simulink subsystem "DCM2quat"  (R2024b)
settings: Solver=VariableStepAuto  StartTime=0.0  StopTime=10.0  RelTol=1e-3
libraries: simulink x2
settings Model: Creator=ferru  LastModifiedBy=domac

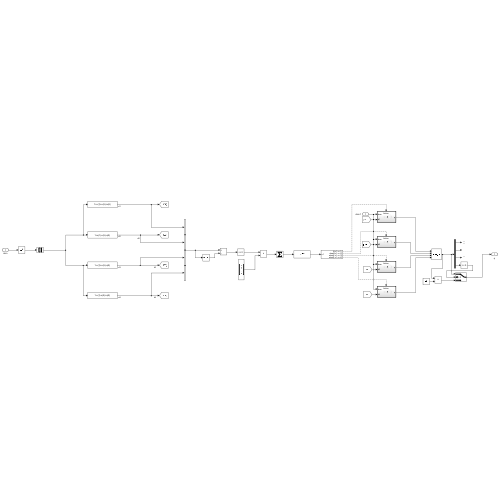
[thumbnail: Simulink's stored preview of the top-level diagram]
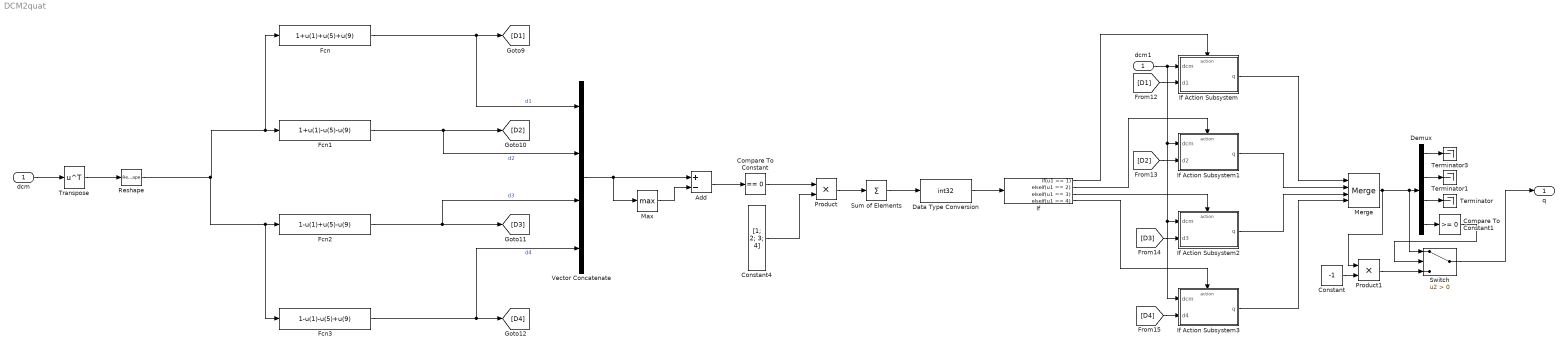
== system DCM2quat ==
  dcm : Inport
  Add : Sum  Inputs=+-
  Compare To Constant : simulink/Logic and Bit Operations/Compare To Constant  relop===  const=0  OutDataTypeStr=boolean
  Compare To Constant1 : simulink/Logic and Bit Operations/Compare To Constant  relop=>=  const=0  OutDataTypeStr=boolean
  Constant : Constant  Value=-1
  Constant4 : Constant  Value=[1; 2; 3; 4]  VectorParams1D=off
  Data Type Conversion : DataTypeConversion  OutDataTypeStr=int32  RndMeth=Round  SaturateOnIntegerOverflow=off
  Demux : Demux
  Fcn : Fcn  Expr=1+u(1)+u(5)+u(9)
  Fcn1 : Fcn  Expr=1+u(1)-u(5)-u(9)
  Fcn2 : Fcn  Expr=1-u(1)+u(5)-u(9)
  Fcn3 : Fcn  Expr=1-u(1)-u(5)+u(9)
  If : If  IfExpression=u1 == 1  ElseIfExpressions=u1 == 2, u1 == 3, u1 == 4  ShowElse=off
  If Action Subsystem : Subsystem  TreatAsAtomicUnit=on
  If Action Subsystem1 : Subsystem  TreatAsAtomicUnit=on
  If Action Subsystem2 : Subsystem  TreatAsAtomicUnit=on
  If Action Subsystem3 : Subsystem  TreatAsAtomicUnit=on
  Max : MinMax  Function=max
  Merge : Merge  Inputs=4
  Product : Product
  Product1 : Product
  Reshape : Reshape  OutputDimensionality=Column vector (2-D)  OutputDimensions=[:,1]
  Sum of Elements : Sum  Inputs=+
  Switch : Switch  Criteria=u2 > Threshold  SaturateOnIntegerOverflow=off  InputSameDT=off
  Terminator : Terminator
  Terminator1 : Terminator
  Terminator3 : Terminator
  Transpose : Math  Operator=transpose
  Vector Concatenate : Concatenate  NumInputs=4
  dcm1 : InportShadow
  q : Outport
  wires:
  dcm/1 -> Transpose/1
  Fcn/1 -> [D1], Vector Concatenate/1  "d1"
  Vector Concatenate/1 -> Max/1, Add/1
  Max/1 -> Add/2
  Add/1 -> Compare To Constant/1
  Product/1 -> Sum of Elements/1
  Constant4/1 -> Product/2
  Compare To Constant/1 -> Product/1
  Sum of Elements/1 -> Data Type Conversion/1
  If/1 -> If Action Subsystem/Action
  If/2 -> If Action Subsystem1/Action
  If/3 -> If Action Subsystem2/Action
  If/4 -> If Action Subsystem3/Action
  dcm1/1 -> If Action Subsystem/1(dcm), If Action Subsystem2/1(dcm), If Action Subsystem3/1(dcm), If Action Subsystem1/1(dcm)
  If Action Subsystem/1(q) -> Merge/1
  If Action Subsystem1/1(q) -> Merge/2
  If Action Subsystem2/1(q) -> Merge/3
  If Action Subsystem3/1(q) -> Merge/4
  Fcn1/1 -> [D2], Vector Concatenate/2  "d2"
  Fcn2/1 -> Vector Concatenate/3, [D3]  "d3"
  Fcn3/1 -> [D4], Vector Concatenate/4  "d4"
  [D1] -> If Action Subsystem/2(d1)
  [D2] -> If Action Subsystem1/2(d2)
  [D3] -> If Action Subsystem2/2(d3)
  [D4] -> If Action Subsystem3/2(d4)
  Reshape/1 -> Fcn1/1, Fcn/1, Fcn2/1, Fcn3/1
  Data Type Conversion/1 -> If/1
  Transpose/1 -> Reshape/1
  Demux/2 -> Terminator1/1
  Demux/3 -> Terminator/1
  Demux/1 -> Terminator3/1
  Merge/1 -> Product1/1, Switch/1, Demux/1
  Demux/4 -> Compare To Constant1/1
  Product1/1 -> Switch/3
  Compare To Constant1/1 -> Switch/2
  Constant/1 -> Product1/2
  Switch/1 -> q/1

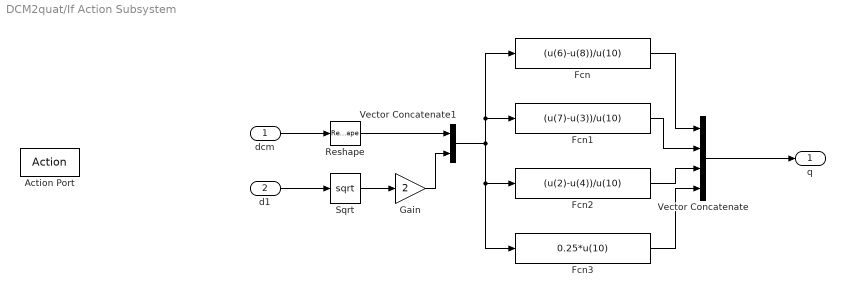
== system DCM2quat/If Action Subsystem ==
  dcm : Inport
  d1 : Inport  Port=2
  Action Port : ActionPort
  Fcn : Fcn  Expr=(u(6)-u(8))/u(10)
  Fcn1 : Fcn  Expr=(u(7)-u(3))/u(10)
  Fcn2 : Fcn  Expr=(u(2)-u(4))/u(10)
  Fcn3 : Fcn  Expr=0.25*u(10)
  Gain : Gain  Gain=2
  Reshape : Reshape  OutputDimensionality=Column vector (2-D)  OutputDimensions=[:,1]
  Sqrt : Sqrt
  Vector Concatenate : Concatenate  NumInputs=4  Mode=Multidimensional array  ConcatenateDimension=2
  Vector Concatenate1 : Concatenate
  q : Outport
  wires:
  Vector Concatenate/1 -> q/1
  Fcn3/1 -> Vector Concatenate/4
  Fcn2/1 -> Vector Concatenate/3
  Fcn1/1 -> Vector Concatenate/2
  Fcn/1 -> Vector Concatenate/1
  Vector Concatenate1/1 -> Fcn1/1, Fcn/1, Fcn3/1, Fcn2/1
  Reshape/1 -> Vector Concatenate1/1
  dcm/1 -> Reshape/1
  Gain/1 -> Vector Concatenate1/2
  Sqrt/1 -> Gain/1
  d1/1 -> Sqrt/1

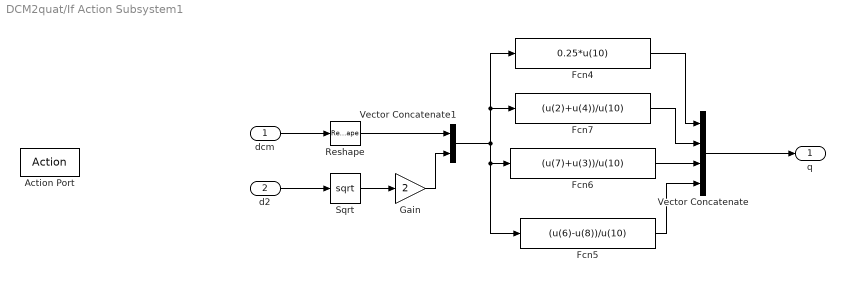
== system DCM2quat/If Action Subsystem1 ==
  dcm : Inport
  d2 : Inport  Port=2
  Action Port : ActionPort
  Fcn4 : Fcn  Expr=0.25*u(10)
  Fcn5 : Fcn  Expr=(u(6)-u(8))/u(10)
  Fcn6 : Fcn  Expr=(u(7)+u(3))/u(10)
  Fcn7 : Fcn  Expr=(u(2)+u(4))/u(10)
  Gain : Gain  Gain=2
  Reshape : Reshape  OutputDimensionality=Column vector (2-D)  OutputDimensions=[:,1]
  Sqrt : Sqrt
  Vector Concatenate : Concatenate  NumInputs=4  Mode=Multidimensional array  ConcatenateDimension=2
  Vector Concatenate1 : Concatenate
  q : Outport
  wires:
  d2/1 -> Sqrt/1
  Sqrt/1 -> Gain/1
  Gain/1 -> Vector Concatenate1/2
  dcm/1 -> Reshape/1
  Reshape/1 -> Vector Concatenate1/1
  Vector Concatenate1/1 -> Fcn6/1, Fcn5/1, Fcn4/1, Fcn7/1
  Fcn4/1 -> Vector Concatenate/1
  Fcn7/1 -> Vector Concatenate/2
  Fcn6/1 -> Vector Concatenate/3
  Fcn5/1 -> Vector Concatenate/4
  Vector Concatenate/1 -> q/1

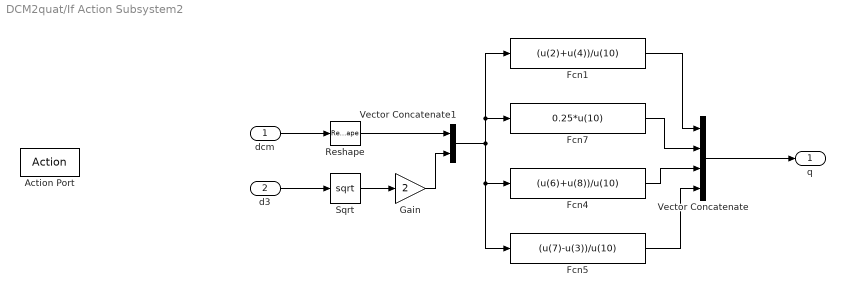
== system DCM2quat/If Action Subsystem2 ==
  dcm : Inport
  d3 : Inport  Port=2
  Action Port : ActionPort
  Fcn1 : Fcn  Expr=(u(2)+u(4))/u(10)
  Fcn4 : Fcn  Expr=(u(6)+u(8))/u(10)
  Fcn5 : Fcn  Expr=(u(7)-u(3))/u(10)
  Fcn7 : Fcn  Expr=0.25*u(10)
  Gain : Gain  Gain=2
  Reshape : Reshape  OutputDimensionality=Column vector (2-D)  OutputDimensions=[:,1]
  Sqrt : Sqrt
  Vector Concatenate : Concatenate  NumInputs=4  Mode=Multidimensional array  ConcatenateDimension=2
  Vector Concatenate1 : Concatenate
  q : Outport
  wires:
  Vector Concatenate/1 -> q/1
  Fcn5/1 -> Vector Concatenate/4
  Fcn4/1 -> Vector Concatenate/3
  Fcn7/1 -> Vector Concatenate/2
  Fcn1/1 -> Vector Concatenate/1
  Vector Concatenate1/1 -> Fcn1/1, Fcn7/1, Fcn4/1, Fcn5/1
  Reshape/1 -> Vector Concatenate1/1
  dcm/1 -> Reshape/1
  Gain/1 -> Vector Concatenate1/2
  Sqrt/1 -> Gain/1
  d3/1 -> Sqrt/1

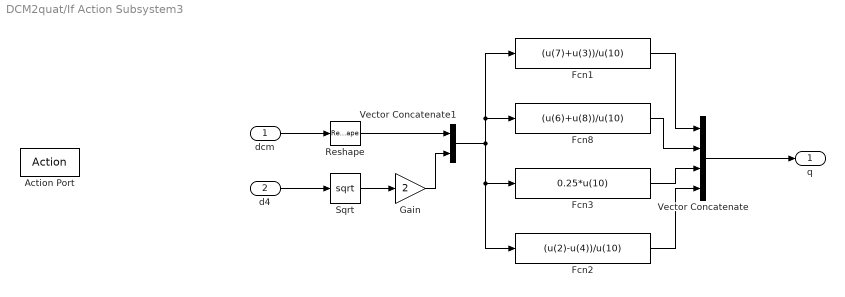
== system DCM2quat/If Action Subsystem3 ==
  dcm : Inport
  d4 : Inport  Port=2
  Action Port : ActionPort
  Fcn1 : Fcn  Expr=(u(7)+u(3))/u(10)
  Fcn2 : Fcn  Expr=(u(2)-u(4))/u(10)
  Fcn3 : Fcn  Expr=0.25*u(10)
  Fcn8 : Fcn  Expr=(u(6)+u(8))/u(10)
  Gain : Gain  Gain=2
  Reshape : Reshape  OutputDimensionality=Column vector (2-D)  OutputDimensions=[:,1]
  Sqrt : Sqrt
  Vector Concatenate : Concatenate  NumInputs=4  Mode=Multidimensional array  ConcatenateDimension=2
  Vector Concatenate1 : Concatenate
  q : Outport
  wires:
  d4/1 -> Sqrt/1
  Sqrt/1 -> Gain/1
  Gain/1 -> Vector Concatenate1/2
  dcm/1 -> Reshape/1
  Reshape/1 -> Vector Concatenate1/1
  Vector Concatenate1/1 -> Fcn3/1, Fcn2/1, Fcn1/1, Fcn8/1
  Fcn1/1 -> Vector Concatenate/1
  Fcn8/1 -> Vector Concatenate/2
  Fcn3/1 -> Vector Concatenate/3
  Fcn2/1 -> Vector Concatenate/4
  Vector Concatenate/1 -> q/1
